simulink model "Simulaciones_Actuadores_Reales"  (R2026b)
settings: Solver=ode15s  StopTime=15  MaxStep=0.001
values from neighbouring files (symbols this model uses):
  alpha_Cu = 3.9e-3    (= 0.0039)    [coeficientes.m]
  b_eq = b_m + b_l/(r^2)    (= 2.19444444444e-05)    [coeficientes.m]
  C_ts = 0.818    [coeficientes.m]
  consigna_p = [0 0 0 0 0 0 0 0 0 0 0 0 ... (16001 elements, 16001x1)]    [perfil_lut.mat]    (also in suavizador_de_consigna.m = p_s(:))
  consigna_t = [0 0.001 0.002 0.003 0.004 0.005 0.006 0.007 0.008 0.009 0.01 0.011 ... (16001 elements, 16001x1)]    [perfil_lut.mat]    (also in suavizador_de_consigna.m = t(:))
  consigna_v = [0 0 0 0 0 0 0 0 0 0 0 0 ... (16001 elements, 16001x1)]    [perfil_lut.mat]    (also in suavizador_de_consigna.m = v_s(:))
  g = 9.80665    [coeficientes.m]
  init_I0 = 0    [coeficientes.m]
  init_Id = 0    [coeficientes.m]
  init_Iq = 0    [coeficientes.m]
  init_theta = 0    [coeficientes.m]
  init_Ts = 20    [coeficientes.m]
  init_w = 0    [coeficientes.m]
  J_eq = J_m + J_l/(r^2)    (= 4.58263888889e-05)    [coeficientes.m]
  K_et = 2*p_obs    (= 6400)    [coeficientes.m]
  K_ew = p_obs^2    (= 10240000)    [coeficientes.m]
  k_l = k_l_min + m_l*l_l    (= 1)    [coeficientes.m]
  Kd_mov = wn_mov * (2*zeta_mov + 1) * J_eq    (= 0.0916527777778)    [coeficientes.m]
  Ki_mov = wn_mov^3 * J_eq    (= 23463.1111111)    [coeficientes.m]
  Kp_mov = wn_mov^2 * (2*zeta_mov + 1) * J_eq    (= 73.3222222222)    [coeficientes.m]
  L_d = 6.6e-3    (= 0.0066)    [coeficientes.m]
  L_ls = 0.8e-3    (= 0.0008)    [coeficientes.m]
  L_q = 5.8e-3    (= 0.0058)    [coeficientes.m]
  lambda = 0.016    [coeficientes.m]
  Pp = 3    [coeficientes.m]
  r = 120.0    (= 120)    [coeficientes.m]
  R0 = abs(p)*L_ls    [coeficientes.m]
  R_sREF = 1.02    [coeficientes.m]
  R_tsamb = 146.7    [coeficientes.m]
  Rd = abs(p)*L_d    [coeficientes.m]
  Rq = abs(p)*L_q    [coeficientes.m]
  sat_V = sqrt(2/3)*V_slMAX    [coeficientes.m]
  T_amb = 20    [coeficientes.m]
  T_sREF = 20    [coeficientes.m]
  tau_RTD = %g s.\n',      base.wn_E,base.wn_I,base.wn_V,base.tau_RTD)    [barrido_filtros_reales.m]    (also in coeficientes.m = 20)
  wn_E = 6000    [coeficientes.m]
  wn_I = 2*6000    (= 12000)    [coeficientes.m]
  wn_V = 8500    [coeficientes.m]
  zeta_E = 1    [coeficientes.m]
  zeta_I = 1    [coeficientes.m]
  zeta_V = 1    [coeficientes.m]
libraries: eeTransforms x5
settings Model: Creator=fedeb  LastModifiedBy=fedeb
settings SimscapeCC: SimscapeLogType=all  SimscapeNominalValues="[{\"value\":\"1\",\"unit\":\"A\"},{\"value\":\"1\",\"unit\":\"bar\"},{\"value\":\"1\",\"unit\":\"cm^2\"},{\"value\":\"1\",\"unit\":\"cm^3/s\"},{\"value\":\"1\",\"unit\":\"kJ/kg\"},{\"value\":\"1\",\"unit\":\"kW\"},{\"value\":\"1\",\"unit\":\"l\"},{\"value\":\"1\",\"unit\":\"N\"},{\"value\":\"1\",\"unit\":\"N*m\"},{\"value\":\"1\",\"unit\":\"V\"},{\"value\":\"0.001\",\"unit\":\"Wb\"}]"  SimscapeUseEnergyAccounting=off

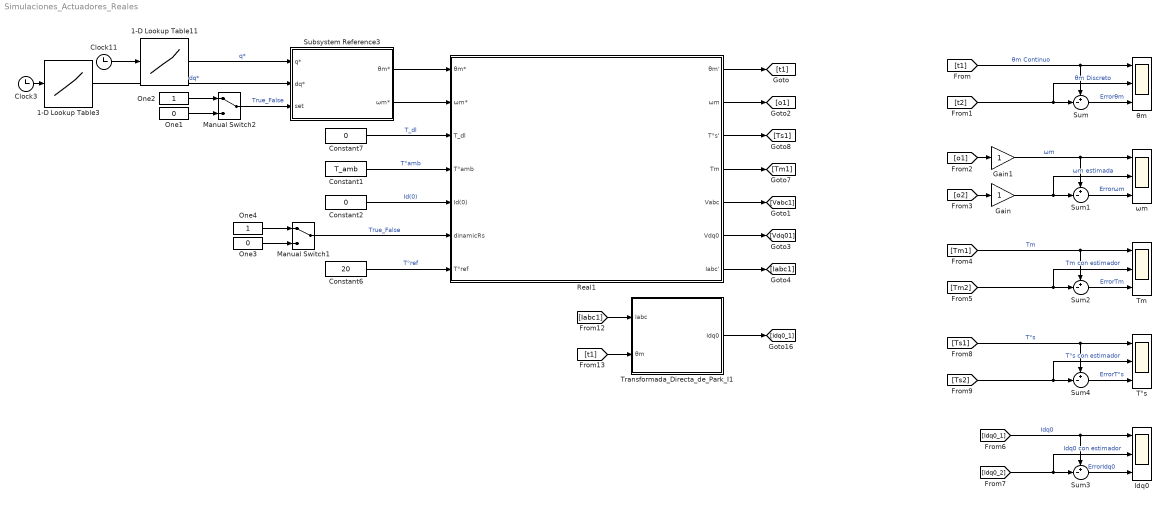
== system Simulaciones_Actuadores_Reales ==
  1-D Lookup Table11 : Lookup_n-D  NumberOfTableDimensions=1  BreakpointsForDimension1=consigna_t  Table=consigna_p  InternalRulePriority=Speed  RndMeth=Simplest
  1-D Lookup Table3 : Lookup_n-D  NumberOfTableDimensions=1  BreakpointsForDimension1=consigna_t  Table=consigna_v  InternalRulePriority=Speed  RndMeth=Simplest
  Clock11 : Clock
  Clock3 : Clock
  Constant1 : Constant  Value=T_amb
  Constant2 : Constant  Value=0
  Constant6 : Constant  Value=20
  Constant7 : Constant  Value=0
  Gain : Gain
  Gain1 : Gain
  Idq0 : Scope  NumInputPorts=3
      settings: Title=Comparación I0 con perturbación  ActiveDisplayYMinimum=-1.47623346288452  ActiveDisplayYMaximum=1.4762334392820955  YLabel=I0 [A]  DataLoggingVariableName=ScopeData3
  Manual Switch1 : ManualSwitch
  Manual Switch2 : ManualSwitch
  One1 : Constant  Value=0  OutDataTypeStr=Inherit: Inherit via back propagation
  One2 : Constant  OutDataTypeStr=Inherit: Inherit via back propagation
  One3 : Constant  Value=0  OutDataTypeStr=Inherit: Inherit via back propagation
  One4 : Constant  OutDataTypeStr=Inherit: Inherit via back propagation
  Real1 : Subsystem
  Subsystem Reference3 : Subsystem
  Sum{,1..4} (5 alike) : Sum  Inputs=+-|
  Tm : Scope  NumInputPorts=3
      settings: Title=Comparación Torque Motor con Perturbacion Tl  ActiveDisplayYMinimum=-0.10628903515783512  ActiveDisplayYMaximum=0.10628903470442332  YLabel=T_m [Nm]
  Transformada_Directa_de_Park_I1 : Subsystem
  T°s : Scope  NumInputPorts=3
      settings: Title=Comparación Temperatura del Estator con Perturbacion Tl  ActiveDisplayYMinimum=-3.1512581688392318  ActiveDisplayYMaximum=28.361323519553096  YLabel=T\circ  DataLoggingVariableName=ScopeData2
  θm : Scope  NumInputPorts=3
      settings: Title=Comparación θ motor con Perturbacion Tl  ActiveDisplayYMinimum=-94.247779700455553  ActiveDisplayYMaximum=848.23001656222721  YLabel=\theta_m[rad]  DataLoggingVariableName=ScopeData4
  ωm : Scope  NumInputPorts=3
      settings: Title=Comparación ωm con Perturbacion Tl  ActiveDisplayYMinimum=-188.49630294307897  ActiveDisplayYMaximum=188.49630291016143  YLabel=\omega_{motor} [10^3 rad/s]  DataLoggingVariableName=ScopeData5
  wires:
  Transformada_Directa_de_Park_I1/1(Idq0) -> [Idq0_1]
  Real1/4(Tm) -> [Tm1]
  Subsystem Reference3/2(ωm*) -> Real1/2(ωm*)
  Constant1/1 -> Real1/4(T°amb)  "T°amb"
  Constant6/1 -> Real1/7(T°ref)  "T°ref"
  Real1/3(T°s') -> [Ts1]
  [t1] -> θm/1, Sum/1  "θm Continuo"
  [Ts1] -> T°s/1, Sum4/1  "T°s"
  [t2] -> θm/2, Sum/2  "θm Discreto"
  Manual Switch2/1 -> Subsystem Reference3/3(set)  "True_False"
  [o2] -> Gain/1
  One3/1 -> Manual Switch1/2
  [Tm2] -> Tm/2, Sum2/2  "Tm con estimador"
  One1/1 -> Manual Switch2/2
  Real1/6(Vdq0) -> [Vdq01]
  Constant7/1 -> Real1/3(T_dl)  "T_dl"
  Gain/1 -> ωm/2, Sum1/2  "ωm estimada"
  Real1/1(θm') -> [t1]
  Subsystem Reference3/1(θm*) -> Real1/1(θm*)
  Real1/5(Vabc) -> [Vabc1]
  Clock3/1 -> 1-D Lookup Table3/1
  1-D Lookup Table11/1 -> Subsystem Reference3/1(q*)  "q*"
  Real1/2(ωm) -> [o1]
  Clock11/1 -> 1-D Lookup Table11/1
  [Ts2] -> T°s/2, Sum4/2  "T°s con estimador"
  Sum3/1 -> Idq0/3  "ErrorIdq0"
  1-D Lookup Table3/1 -> Subsystem Reference3/2(dq*)  "dq*"
  [Tm1] -> Tm/1, Sum2/1  "Tm"
  One2/1 -> Manual Switch2/1
  Sum4/1 -> T°s/3  "ErrorT°s"
  Constant2/1 -> Real1/5(Id(0))  "Id(0)"
  Sum2/1 -> Tm/3  "ErrorTm"
  [o1] -> Gain1/1
  [t1] -> Transformada_Directa_de_Park_I1/2(θm)
  Real1/7(Iabc') -> [Iabc1]
  [Idq0_2] -> Idq0/2, Sum3/2  "Idq0 con estimador"
  [Idq0_1] -> Sum3/1, Idq0/1  "Idq0"
  [Iabc1] -> Transformada_Directa_de_Park_I1/1(Iabc)
  Manual Switch1/1 -> Real1/6(dinamicRs)  "True_False"
  Sum/1 -> θm/3  "Errorθm"
  One4/1 -> Manual Switch1/1
  Sum1/1 -> ωm/3  "Errorωm"
  Gain1/1 -> ωm/1, Sum1/1  "ωm"

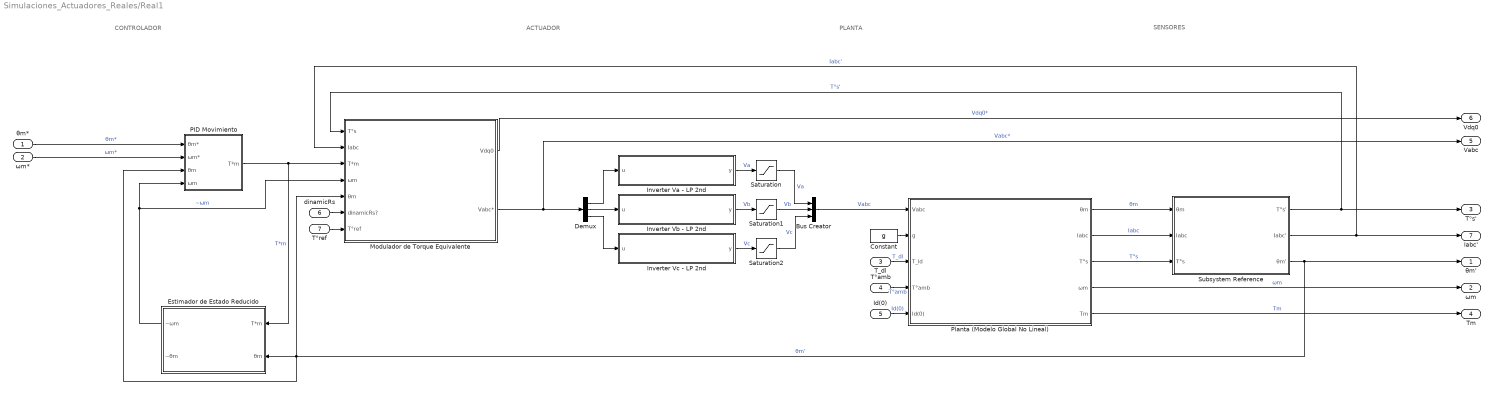
== system Simulaciones_Actuadores_Reales/Real1 ==
  note: ACTUADOR
  note: SENSORES
  note: CONTROLADOR
  note: PLANTA
  θm* : Inport
  ωm* : Inport  Port=2
  T_dl : Inport  Port=3
  T°amb : Inport  Port=4
  Id(0) : Inport  Port=5
  dinamicRs : Inport  Port=6
  T°ref : Inport  Port=7
  Bus Creator : BusCreator  Inputs=3
  Constant : Constant  Value=g
  Demux : Demux  Outputs=3
  Estimador de Estado Reducido : Subsystem
  Inverter Va - LP 2nd : Subsystem
  Inverter Vb - LP 2nd : Subsystem
  Inverter Vc - LP 2nd : Subsystem
  Modulador de Torque Equivalente : Subsystem
      settings: PortSchema="{\"entries\":[{\"content\":{\"sides\":[{\"content\":{\"connectorIds\":[\"In1\",\"In3\",\"In5\",\"In2\",\"In4\",\"In6\",\"In7\"]},\"type\":\"ConnectorPlacement.EquallySpacedRectSide\",\"uuid\":\"ea9ad4ab-f607-4d37-9442-85f6cfda2486\"},{\"content\":{\"connectorIds\":[\"Out2\",\"Out1\"],\"side\":\"RIGHT\"},\"type\":\"ConnectorPlacement.EquallySpacedRectSide\",\"uuid\":\"696b5fe5-1f6c-4fc9-932e-86b56d49996f\"},{\"content\":{\"side\":\"TOP\"},\"type\":\"ConnectorPlacement.EquallySpacedRectSide\",\"uuid\":\"45e3ac4c-5a2f-4a79-9454-e497b07295c7\"}]},\"type\":\"ConnectorPlacement.EquallySpacedConnector\",\"uuid\":\"ad401c21-3c60-4ab4-96eb-f449fc93609a\"}],\"packageUris\":[\"http://schema.mathworks.com/mf0/Connector/R2020b\"],\"version\":\"1.0\"}"
  PID Movimiento : Subsystem
      settings: PortSchema="{\"entries\":[{\"content\":{\"sides\":[{\"content\":{\"connectorIds\":[\"In3\",\"In4\",\"In2\",\"In1\"]},\"type\":\"ConnectorPlacement.EquallySpacedRectSide\",\"uuid\":\"99b9ec4b-f651-40ed-8a16-085c2c4ac88d\"},{\"content\":{\"connectorIds\":[\"Out1\"],\"side\":\"RIGHT\"},\"type\":\"ConnectorPlacement.EquallySpacedRectSide\",\"uuid\":\"009a9369-fd86-4ac2-a423-7c7f1491457b\"},{\"content\":{\"side\":\"TOP\"},\"type\":\"ConnectorPlacement.EquallySpacedRectSide\",\"uuid\":\"0bc889a5-9100-482e-a11a-4c36993d76f7\"}]},\"type\":\"ConnectorPlacement.EquallySpacedConnector\",\"uuid\":\"de270b8a-8a15-46e7-87f3-10db7988a399\"}],\"packageUris\":[\"http://schema.mathworks.com/mf0/Connector/R2020b\"],\"version\":\"1.0\"}"
  Planta (Modelo Global No Lineal) : Subsystem
      settings: PortSchema="{\"entries\":[{\"content\":{\"sides\":[{\"content\":{\"connectorIds\":[\"In1\",\"In3\",\"In2\",\"In4\",\"In5\"]},\"type\":\"ConnectorPlacement.EquallySpacedRectSide\",\"uuid\":\"3481abf0-b0cb-49f6-b93f-5a31fbfa4119\"},{\"content\":{\"connectorIds\":[\"Out1\",\"Out2\",\"Out3\",\"Out4\",\"Out5\"],\"side\":\"RIGHT\"},\"type\":\"ConnectorPlacement.EquallySpacedRectSide\",\"uuid\":\"81dbc61e-d5f3-4edc-bc73-ec3d6160a008\"},{\"content\":{\"side\":\"TOP\"},\"type\":\"ConnectorPlacement.EquallySpacedRectSide\",\"uuid\":\"48e37594-92fb-4835-b4aa-9211b8b6a309\"}]},\"type\":\"ConnectorPlacement.EquallySpacedConnector\",\"uuid\":\"6c32b8e1-5803-41f4-af4e-ba3a494349ba\"}],\"packageUris\":[\"http://schema.mathworks.com/mf0/Connector/R2020b\"],\"version\":\"1.0\"}"
  Saturation : Saturate  UpperLimit=sat_V  LowerLimit=-sat_V
  Saturation1 : Saturate  UpperLimit=sat_V  LowerLimit=-sat_V
  Saturation2 : Saturate  UpperLimit=sat_V  LowerLimit=-sat_V
  Subsystem Reference : Subsystem
  θm' : Outport
  ωm : Outport  Port=2
  T°s' : Outport  Port=3
  Tm : Outport  Port=4
  Vabc : Outport  Port=5  OutDataTypeStr=Bus: Vabc
  Vdq0 : Outport  Port=6  OutDataTypeStr=Bus: Vdq0
  Iabc' : Outport  Port=7  OutDataTypeStr=Bus: Iabc
  wires:
  Subsystem Reference/2(Iabc') -> Modulador de Torque Equivalente/3(Iabc), Iabc'/1  "Iabc'"
  Planta (Modelo Global No Lineal)/2(Iabc) -> Subsystem Reference/2(Iabc)  "Iabc"
  T°amb/1 -> Planta (Modelo Global No Lineal)/4(T°amb)  "T°amb"
  T°ref/1 -> Modulador de Torque Equivalente/7(T°ref)
  T_dl/1 -> Planta (Modelo Global No Lineal)/2(T_ld)  "T_dl"
  Subsystem Reference/1(T°s') -> Modulador de Torque Equivalente/1(T°s), T°s'/1  "T°s'"
  dinamicRs/1 -> Modulador de Torque Equivalente/6(dinamicRs?)
  Planta (Modelo Global No Lineal)/5(Tm) -> Tm/1  "Tm"
  θm*/1 -> PID Movimiento/3(θm*)  "θm*"
  Modulador de Torque Equivalente/2(Vdq0) -> Vdq0/1  "Vdq0*"
  Planta (Modelo Global No Lineal)/4(ωm) -> ωm/1  "ωm"
  PID Movimiento/1(T*m) -> Estimador de Estado Reducido/1(T*m), Modulador de Torque Equivalente/5(T*m)  "T*m"
  Estimador de Estado Reducido/1(~ωm) -> PID Movimiento/1(ωm), Modulador de Torque Equivalente/2(ωm)  "~ωm"
  Constant/1 -> Planta (Modelo Global No Lineal)/3(g)
  ωm*/1 -> PID Movimiento/4(ωm*)  "ωm*"
  Planta (Modelo Global No Lineal)/1(θm) -> Subsystem Reference/1(θm)  "θm"
  Id(0)/1 -> Planta (Modelo Global No Lineal)/5(Id(0))  "Id(0)"
  Subsystem Reference/3(θm') -> Modulador de Torque Equivalente/4(θm), PID Movimiento/2(θm), Estimador de Estado Reducido/2(θm), θm'/1  "θm'"
  Planta (Modelo Global No Lineal)/3(T°s) -> Subsystem Reference/3(T°s)  "T°s"
  Demux/2 -> Inverter Vb - LP 2nd/1(u)
  Inverter Vc - LP 2nd/1(y) -> Saturation2/1  "Vc"
  Saturation1/1 -> Bus Creator/2  "Vb"
  Inverter Vb - LP 2nd/1(y) -> Saturation1/1  "Vb"
  Demux/1 -> Inverter Va - LP 2nd/1(u)
  Inverter Va - LP 2nd/1(y) -> Saturation/1  "Va"
  Demux/3 -> Inverter Vc - LP 2nd/1(u)
  Modulador de Torque Equivalente/1(Vabc*) -> Demux/1, Vabc/1  "Vabc*"
  Saturation2/1 -> Bus Creator/3  "Vc"
  Bus Creator/1 -> Planta (Modelo Global No Lineal)/1(Vabc)  "Vabc"
  Saturation/1 -> Bus Creator/1  "Va"

== system Simulaciones_Actuadores_Reales/Subsystem Reference3 ==
  q* : Inport
  dq* : Inport  Port=2
  set : Inport  Port=3
  Gain : Gain  Gain=r
  Gain1 : Gain  Gain=r
  Integrator : Integrator  ExternalReset=level  InitialConditionSource=external
  Selector : RelationalOperator  Operator=>  OutDataTypeStr=boolean  RndMeth=Simplest  InputSameDT=off
  Switch : Switch  Criteria=u2 ~= 0  SaturateOnIntegerOverflow=off  InputSameDT=off
  Umbral : Constant  Value=0.5
  θm* : Outport
  ωm* : Outport  Port=2
  wires:
  q*/1 -> Gain/1
  dq*/1 -> Gain1/1
  set/1 -> Selector/1
  Umbral/1 -> Selector/2
  Gain/1 -> Integrator/3, Switch/1
  Selector/1 -> Integrator/2, Switch/2
  Gain1/1 -> Integrator/1, ωm*/1
  Integrator/1 -> Switch/3
  Switch/1 -> θm*/1

== system Simulaciones_Actuadores_Reales/Transformada_Directa_de_Park_I1 ==
  Iabc : Inport  OutDataTypeStr=Bus: Iabc
  θm : Inport  Port=2
  Ancho_abc : SignalSpecification  Dimensions=3
  Bus Creator : BusCreator  Inputs=3
  Bus to Vector : BusToVector
  Demux : Demux  Outputs=3
  Gain3 : Gain  Gain=Pp
  Park Transform : eeTransforms/Park Transform  AxisAlignment=Q-axis  PowerInvariant=off
      settings: LibrarySourceBlock=|
      | ee_sl_lib/Mathematical
      | Transforms/Park Transform
  Idq0 : Outport  OutDataTypeStr=Bus: Idq0
  wires:
  Gain3/1 -> Park Transform/2
  Park Transform/1 -> Demux/1  "Idq0"
  Demux/1 -> Bus Creator/1  "Id"
  Demux/3 -> Bus Creator/3  "I0"
  Demux/2 -> Bus Creator/2  "Iq"
  Bus Creator/1 -> Idq0/1
  Iabc/1 -> Bus to Vector/1
  θm/1 -> Gain3/1
  Bus to Vector/1 -> Ancho_abc/1
  Ancho_abc/1 -> Park Transform/1

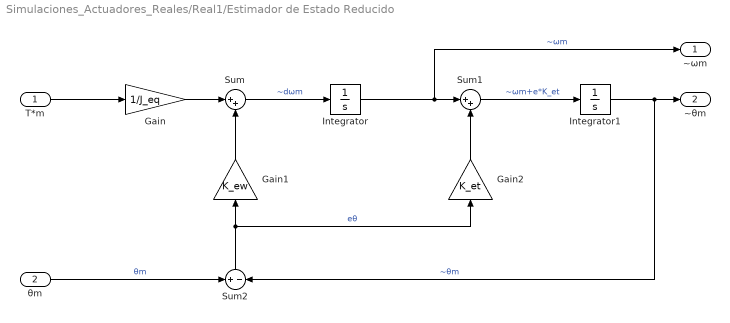
== system Simulaciones_Actuadores_Reales/Real1/Estimador de Estado Reducido ==
  T*m : Inport
  θm : Inport  Port=2
  Gain : Gain  Gain=1/J_eq
  Gain1 : Gain  Gain=K_ew
  Gain2 : Gain  Gain=K_et
  Integrator : Integrator
  Integrator1 : Integrator
  Sum : Sum  Inputs=|++
  Sum1 : Sum  Inputs=|++
  Sum2 : Sum  Inputs=+-
  ~ωm : Outport
  ~θm : Outport  Port=2
  wires:
  Integrator1/1 -> ~θm/1, Sum2/2  "~θm"
  θm/1 -> Sum2/1  "θm"
  Sum2/1 -> Gain2/1, Gain1/1  "eθ"
  Gain2/1 -> Sum1/2
  Gain1/1 -> Sum/2
  Integrator/1 -> Sum1/1, ~ωm/1  "~ωm"
  Sum1/1 -> Integrator1/1  "~ωm+e*K_et"
  Sum/1 -> Integrator/1  "~dωm"
  Gain/1 -> Sum/1
  T*m/1 -> Gain/1

== system Simulaciones_Actuadores_Reales/Real1/Inverter Va - LP 2nd ==
  u : Inport
  Gain : Gain  Gain=wn_V^2
  Gain1 : Gain  Gain=wn_V^2
  Gain2 : Gain  Gain=2*zeta_V*wn_V
  Integrator : Integrator
  Integrator1 : Integrator
  Sum : Sum  Inputs=|++
  Sum1 : Sum  Inputs=|+-
  y : Outport
  wires:
  u/1 -> Gain/1
  Gain/1 -> Sum1/1
  Sum/1 -> Sum1/2
  Sum1/1 -> Integrator/1
  Gain2/1 -> Sum/2
  Gain1/1 -> Sum/1
  Integrator/1 -> Gain2/1, Integrator1/1
  Integrator1/1 -> Gain1/1, y/1

== system Simulaciones_Actuadores_Reales/Real1/Inverter Vb - LP 2nd ==
  u : Inport
  Gain : Gain  Gain=wn_V^2
  Gain1 : Gain  Gain=wn_V^2
  Gain2 : Gain  Gain=2*zeta_V*wn_V
  Integrator : Integrator
  Integrator1 : Integrator
  Sum : Sum  Inputs=|++
  Sum1 : Sum  Inputs=|+-
  y : Outport
  wires:
  Integrator1/1 -> y/1, Gain1/1
  Integrator/1 -> Integrator1/1, Gain2/1
  Gain1/1 -> Sum/1
  Gain2/1 -> Sum/2
  Sum1/1 -> Integrator/1
  Sum/1 -> Sum1/2
  Gain/1 -> Sum1/1
  u/1 -> Gain/1

== system Simulaciones_Actuadores_Reales/Real1/Inverter Vc - LP 2nd ==
  u : Inport
  Gain : Gain  Gain=wn_V^2
  Gain1 : Gain  Gain=wn_V^2
  Gain2 : Gain  Gain=2*zeta_V*wn_V
  Integrator : Integrator
  Integrator1 : Integrator
  Sum : Sum  Inputs=|++
  Sum1 : Sum  Inputs=|+-
  y : Outport
  wires:
  u/1 -> Gain/1
  Gain/1 -> Sum1/1
  Sum/1 -> Sum1/2
  Sum1/1 -> Integrator/1
  Gain2/1 -> Sum/2
  Gain1/1 -> Sum/1
  Integrator/1 -> Gain2/1, Integrator1/1
  Integrator1/1 -> Gain1/1, y/1

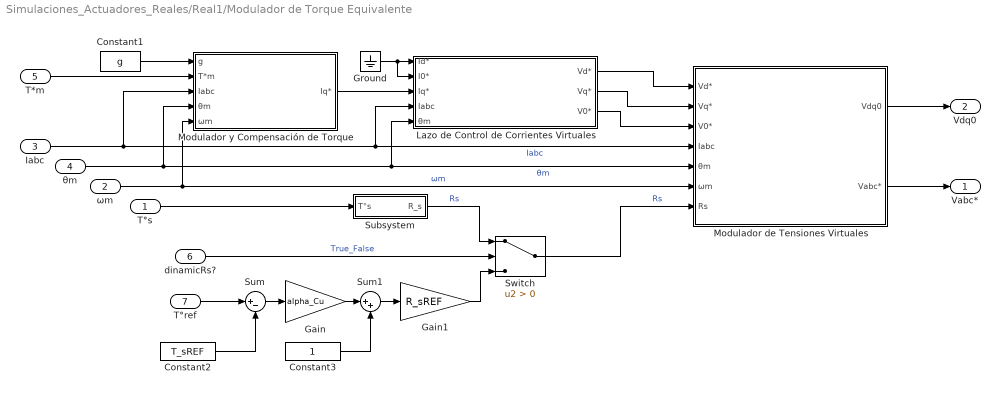
== system Simulaciones_Actuadores_Reales/Real1/Modulador de Torque Equivalente ==
  T°s : Inport
  ωm : Inport  Port=2
  Iabc : Inport  Port=3
  θm : Inport  Port=4
  T*m : Inport  Port=5
  dinamicRs? : Inport  Port=6
  T°ref : Inport  Port=7
  Constant1 : Constant  Value=g
  Constant2 : Constant  Value=T_sREF
  Constant3 : Constant
  Gain : Gain  Gain=alpha_Cu
  Gain1 : Gain  Gain=R_sREF
  Ground : Ground
  Lazo de Control de Corrientes Virtuales : Subsystem
      settings: PortSchema="{\"entries\":[{\"content\":{\"sides\":[{\"content\":{\"connectorIds\":[\"In2\",\"In3\",\"In1\",\"In4\",\"In5\"]},\"type\":\"ConnectorPlacement.EquallySpacedRectSide\",\"uuid\":\"7378df2b-1b9c-42cd-9ef6-9bfa4de31228\"},{\"content\":{\"connectorIds\":[\"Out2\",\"Out1\",\"Out3\"],\"side\":\"RIGHT\"},\"type\":\"ConnectorPlacement.EquallySpacedRectSide\",\"uuid\":\"75ac4e09-b611-4ee2-aa1e-16791f3f98b8\"},{\"content\":{\"side\":\"TOP\"},\"type\":\"ConnectorPlacement.EquallySpacedRectSide\",\"uuid\":\"c32b7829-5b6a-417b-8aae-eaa4caf59bef\"}]},\"type\":\"ConnectorPlacement.EquallySpacedConnector\",\"uuid\":\"1d84f5ff-db01-492a-bfe1-22065b3eebb0\"}],\"packageUris\":[\"http://schema.mathworks.com/mf0/Connector/R2020b\"],\"version\":\"1.0\"}"
  Modulador de Tensiones Virtuales : Subsystem
      settings: PortSchema="{\"entries\":[{\"content\":{\"sides\":[{\"content\":{\"connectorIds\":[\"In2\",\"In1\",\"In3\",\"In6\",\"In7\",\"In5\",\"In4\"]},\"type\":\"ConnectorPlacement.EquallySpacedRectSide\",\"uuid\":\"561a625a-719f-47d4-85d3-a88e423068dd\"},{\"content\":{\"connectorIds\":[\"Out2\",\"Out1\"],\"side\":\"RIGHT\"},\"type\":\"ConnectorPlacement.EquallySpacedRectSide\",\"uuid\":\"c1cdd74a-6c1d-470e-a6ac-8d72e83b5cc5\"},{\"content\":{\"side\":\"TOP\"},\"type\":\"ConnectorPlacement.EquallySpacedRectSide\",\"uuid\":\"c5935c6f-534c-46b9-aa64-6d6dabbbb210\"}]},\"type\":\"ConnectorPlacement.EquallySpacedConnector\",\"uuid\":\"b0debde9-6e18-4e06-b0c4-28c9c51e472d\"}],\"packageUris\":[\"http://schema.mathworks.com/mf0/Connector/R2020b\"],\"version\":\"1.0\"}"
  Modulador y Compensación de Torque : Subsystem
      settings: PortSchema="{\"entries\":[{\"content\":{\"sides\":[{\"content\":{\"connectorIds\":[\"In5\",\"In1\",\"In2\",\"In3\",\"In4\"]},\"type\":\"ConnectorPlacement.EquallySpacedRectSide\",\"uuid\":\"ea9ad4ab-f607-4d37-9442-85f6cfda2486\"},{\"content\":{\"connectorIds\":[\"Out1\"],\"side\":\"RIGHT\"},\"type\":\"ConnectorPlacement.EquallySpacedRectSide\",\"uuid\":\"696b5fe5-1f6c-4fc9-932e-86b56d49996f\"},{\"content\":{\"side\":\"TOP\"},\"type\":\"ConnectorPlacement.EquallySpacedRectSide\",\"uuid\":\"45e3ac4c-5a2f-4a79-9454-e497b07295c7\"}]},\"type\":\"ConnectorPlacement.EquallySpacedConnector\",\"uuid\":\"ad401c21-3c60-4ab4-96eb-f449fc93609a\"}],\"packageUris\":[\"http://schema.mathworks.com/mf0/Connector/R2020b\"],\"version\":\"1.0\"}"
  Subsystem : Subsystem
  Sum : Sum  Inputs=|+-
  Sum1 : Sum  Inputs=|++
  Switch : Switch  Criteria=u2 > Threshold  SaturateOnIntegerOverflow=off  InputSameDT=off
  Vabc* : Outport
  Vdq0 : Outport  Port=2
  wires:
  Sum1/1 -> Gain1/1
  Constant3/1 -> Sum1/2
  Gain/1 -> Sum1/1
  Sum/1 -> Gain/1
  Constant2/1 -> Sum/2
  T°ref/1 -> Sum/1
  Constant1/1 -> Modulador y Compensación de Torque/5(g)
  Modulador de Tensiones Virtuales/2(Vdq0) -> Vdq0/1
  Gain1/1 -> Switch/3
  Switch/1 -> Modulador de Tensiones Virtuales/4(Rs)  "Rs"
  dinamicRs?/1 -> Switch/2  "True_False"
  Subsystem/1(R_s) -> Switch/1  "Rs"
  T°s/1 -> Subsystem/1(T°s)
  Iabc/1 -> Modulador y Compensación de Torque/2(Iabc), Lazo de Control de Corrientes Virtuales/4(Iabc), Modulador de Tensiones Virtuales/6(Iabc)  "Iabc"
  Ground/1 -> Lazo de Control de Corrientes Virtuales/3(I0*), Lazo de Control de Corrientes Virtuales/2(Id*)
  Modulador de Tensiones Virtuales/1(Vabc*) -> Vabc*/1
  ωm/1 -> Modulador y Compensación de Torque/4(ωm), Modulador de Tensiones Virtuales/5(ωm)  "ωm"
  θm/1 -> Modulador y Compensación de Torque/3(θm), Lazo de Control de Corrientes Virtuales/5(θm), Modulador de Tensiones Virtuales/7(θm)  "θm"
  T*m/1 -> Modulador y Compensación de Torque/1(T*m)
  Modulador y Compensación de Torque/1(Iq*) -> Lazo de Control de Corrientes Virtuales/1(Iq*)
  Lazo de Control de Corrientes Virtuales/3(V0*) -> Modulador de Tensiones Virtuales/3(V0*)
  Lazo de Control de Corrientes Virtuales/2(Vd*) -> Modulador de Tensiones Virtuales/2(Vd*)
  Lazo de Control de Corrientes Virtuales/1(Vq*) -> Modulador de Tensiones Virtuales/1(Vq*)

== system Simulaciones_Actuadores_Reales/Real1/PID Movimiento ==
  ωm : Inport  Unit=rad/s
  θm : Inport  Port=2
  θm* : Inport  Port=3  Unit=rad/s
  ωm* : Inport  Port=4  Unit=rad/s
  Gain : Gain  Gain=Kd_mov
  Gain1 : Gain  Gain=Kp_mov
  Gain2 : Gain  Gain=Ki_mov
  Integrator : Integrator
  Sum : Sum  Inputs=|+-
  Sum1 : Sum  Inputs=+++
  Sum2 : Sum  Inputs=|+-
  T*m : Outport
  wires:
  Sum2/1 -> Integrator/1, Gain1/1  "eθ"
  Integrator/1 -> Gain2/1  "e∫θ"
  ωm/1 -> Sum/2
  ωm*/1 -> Sum/1
  θm/1 -> Sum2/2
  Sum/1 -> Gain/1  "eω"
  θm*/1 -> Sum2/1
  Gain/1 -> Sum1/3
  Gain2/1 -> Sum1/1
  Sum1/1 -> T*m/1
  Gain1/1 -> Sum1/2

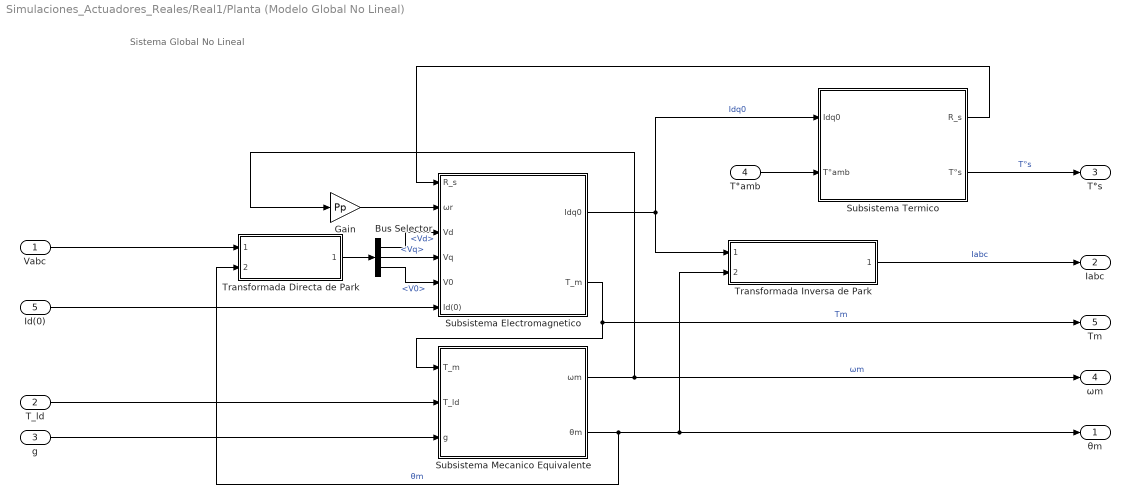
== system Simulaciones_Actuadores_Reales/Real1/Planta (Modelo Global No Lineal) ==
  note: Sistema Global No Lineal
  Vabc : Inport  OutDataTypeStr=Bus: Vabc
  T_ld : Inport  Port=2
  g : Inport  Port=3
  T°amb : Inport  Port=4
  Id(0) : Inport  Port=5
  Bus Selector : BusSelector  OutputSignals=Vd,Vq,V0
  Gain : Gain  Gain=Pp
  Subsistema Electromagnetico : Subsystem
  Subsistema Mecanico Equivalente : Subsystem
  Subsistema Termico : Subsystem
  Transformada Directa de Park : Subsystem  ReferencedSubsystem=Transformada_Directa_de_Park_V
  Transformada Inversa de Park : Subsystem  ReferencedSubsystem=Transformada_Inversa_de_Park_I
  θm : Outport
  Iabc : Outport  Port=2  OutDataTypeStr=Bus: Iabc
  T°s : Outport  Port=3
  ωm : Outport  Port=4
  Tm : Outport  Port=5
  wires:
  Id(0)/1 -> Subsistema Electromagnetico/6(Id(0))
  Transformada Inversa de Park/1 -> Iabc/1  "Iabc"
  Bus Selector/3 -> Subsistema Electromagnetico/5(V0)  "<V0>"
  Bus Selector/2 -> Subsistema Electromagnetico/4(Vq)  "<Vq>"
  Bus Selector/1 -> Subsistema Electromagnetico/3(Vd)  "<Vd>"
  Transformada Directa de Park/1 -> Bus Selector/1
  g/1 -> Subsistema Mecanico Equivalente/3(g)
  T°amb/1 -> Subsistema Termico/2(T°amb)
  Vabc/1 -> Transformada Directa de Park/1
  T_ld/1 -> Subsistema Mecanico Equivalente/2(T_ld)
  Gain/1 -> Subsistema Electromagnetico/2(ωr)
  Subsistema Termico/1(R_s) -> Subsistema Electromagnetico/1(R_s)
  Subsistema Electromagnetico/2(T_m) -> Tm/1, Subsistema Mecanico Equivalente/1(T_m)  "Tm"
  Subsistema Mecanico Equivalente/2(θm) -> θm/1, Transformada Inversa de Park/2, Transformada Directa de Park/2  "θm"
  Subsistema Mecanico Equivalente/1(ωm) -> ωm/1, Gain/1  "ωm"
  Subsistema Electromagnetico/1(Idq0) -> Transformada Inversa de Park/1, Subsistema Termico/1(Idq0)  "Idq0"
  Subsistema Termico/2(T°s) -> T°s/1  "T°s"

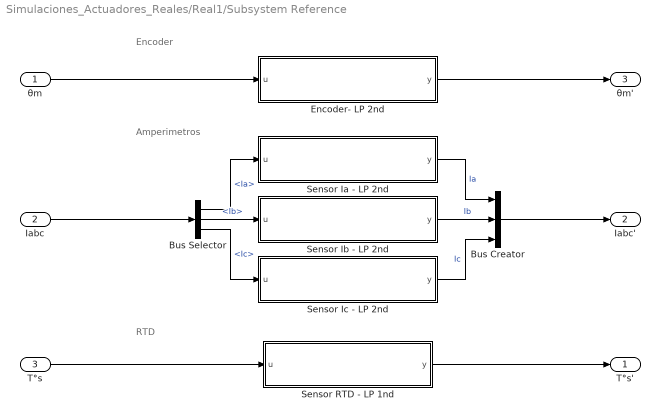
== system Simulaciones_Actuadores_Reales/Real1/Subsystem Reference ==
  note: Amperimetros
  note: Encoder
  note: RTD
  θm : Inport
  Iabc : Inport  Port=2
  T°s : Inport  Port=3
  Bus Creator : BusCreator  Inputs=3
  Bus Selector : BusSelector  OutputSignals=Ia,Ib,Ic
  Encoder- LP 2nd : Subsystem
  Sensor Ia - LP 2nd : Subsystem
  Sensor Ib - LP 2nd : Subsystem
  Sensor Ic - LP 2nd : Subsystem
  Sensor RTD - LP 1nd : Subsystem
  T°s' : Outport
  Iabc' : Outport  Port=2
  θm' : Outport  Port=3
  wires:
  Sensor Ib - LP 2nd/1(y) -> Bus Creator/2  "Ib"
  Sensor RTD - LP 1nd/1(y) -> T°s'/1
  Sensor Ia - LP 2nd/1(y) -> Bus Creator/1  "Ia"
  Bus Creator/1 -> Iabc'/1
  Encoder- LP 2nd/1(y) -> θm'/1
  Bus Selector/1 -> Sensor Ia - LP 2nd/1(u)  "<Ia>"
  Bus Selector/2 -> Sensor Ib - LP 2nd/1(u)  "<Ib>"
  T°s/1 -> Sensor RTD - LP 1nd/1(u)
  Bus Selector/3 -> Sensor Ic - LP 2nd/1(u)  "<Ic>"
  Iabc/1 -> Bus Selector/1
  θm/1 -> Encoder- LP 2nd/1(u)
  Sensor Ic - LP 2nd/1(y) -> Bus Creator/3  "Ic"

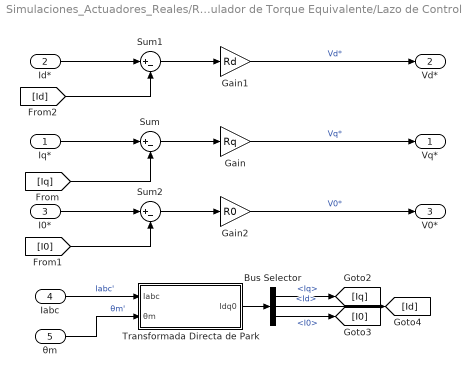
== system Simulaciones_Actuadores_Reales/Real1/Modulador de Torque Equivalente/Lazo de Control de Corrientes Virtuales ==
  Iq* : Inport
  Id* : Inport  Port=2
  I0* : Inport  Port=3
  Iabc : Inport  Port=4
  θm : Inport  Port=5
  Bus Selector : BusSelector  OutputSignals=Iq,Id,I0
  Gain : Gain  Gain=Rq
  Gain1 : Gain  Gain=Rd
  Gain2 : Gain  Gain=R0
  Sum : Sum  Inputs=|+-
  Sum1 : Sum  Inputs=|+-
  Sum2 : Sum  Inputs=|+-
  Transformada Directa de Park : Subsystem
  Vq* : Outport
  Vd* : Outport  Port=2
  V0* : Outport  Port=3
  wires:
  Sum1/1 -> Gain1/1
  Gain/1 -> Vq*/1  "Vq*"
  Id*/1 -> Sum1/1
  Iq*/1 -> Sum/1
  Gain1/1 -> Vd*/1  "Vd*"
  [Iq] -> Sum/2
  [Id] -> Sum1/2
  Sum/1 -> Gain/1
  Gain2/1 -> V0*/1  "V0*"
  Sum2/1 -> Gain2/1
  [I0] -> Sum2/2
  I0*/1 -> Sum2/1
  Bus Selector/2 -> [Id]  "<Id>"
  Bus Selector/3 -> [I0]  "<I0>"
  Transformada Directa de Park/1(Idq0) -> Bus Selector/1
  Iabc/1 -> Transformada Directa de Park/1(Iabc)  "Iabc'"
  θm/1 -> Transformada Directa de Park/2(θm)  "θm'"
  Bus Selector/1 -> [Iq]  "<Iq>"

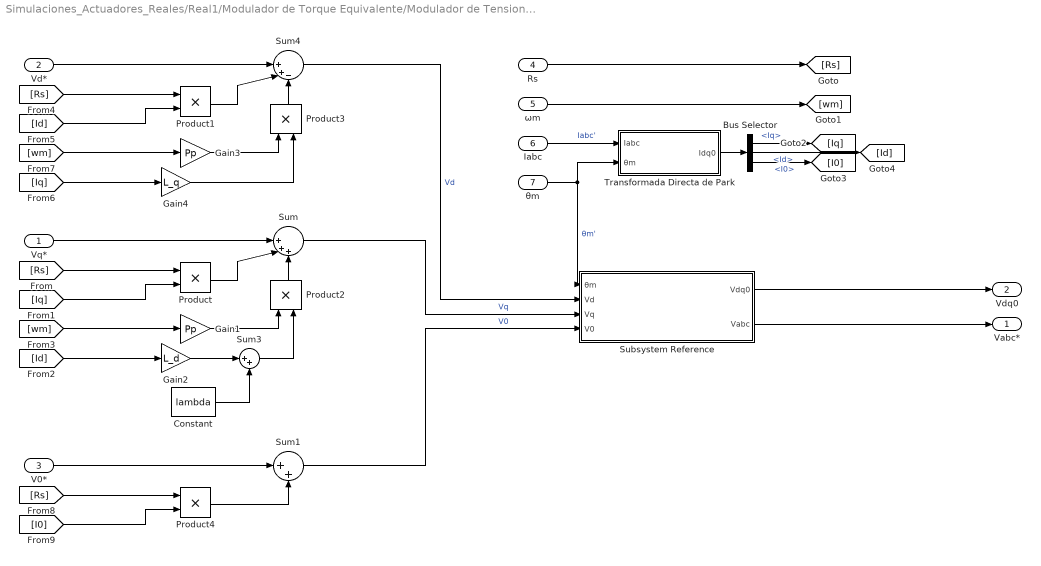
== system Simulaciones_Actuadores_Reales/Real1/Modulador de Torque Equivalente/Modulador de Tensiones Virtuales ==
  Vq* : Inport
  Vd* : Inport  Port=2
  V0* : Inport  Port=3
  Rs : Inport  Port=4
  ωm : Inport  Port=5
  Iabc : Inport  Port=6
  θm : Inport  Port=7
  Bus Selector : BusSelector  OutputSignals=Iq,Id,I0
  Constant : Constant  Value=lambda
  Gain1 : Gain  Gain=Pp
  Gain2 : Gain  Gain=L_d
  Gain3 : Gain  Gain=Pp
  Gain4 : Gain  Gain=L_q
  Product{,1..4} (5 alike) : Product
  Subsystem Reference : Subsystem
  Sum : Sum  Inputs=||+++
  Sum1 : Sum  Inputs=|++
  Sum3 : Sum  Inputs=|++
  Sum4 : Sum  Inputs=||++-
  Transformada Directa de Park : Subsystem
  Vabc* : Outport
  Vdq0 : Outport  Port=2
  wires:
  Sum1/1 -> Subsystem Reference/4(V0)  "V0"
  Sum/1 -> Subsystem Reference/3(Vq)  "Vq"
  Sum4/1 -> Subsystem Reference/2(Vd)  "Vd"
  Subsystem Reference/1(Vdq0) -> Vdq0/1
  Iabc/1 -> Transformada Directa de Park/1(Iabc)  "Iabc'"
  Transformada Directa de Park/1(Idq0) -> Bus Selector/1
  θm/1 -> Transformada Directa de Park/2(θm), Subsystem Reference/1(θm)  "θm'"
  Subsystem Reference/2(Vabc) -> Vabc*/1
  Rs/1 -> [Rs]
  ωm/1 -> [wm]
  Bus Selector/1 -> [Iq]  "<Iq>"
  Bus Selector/3 -> [I0]  "<I0>"
  Bus Selector/2 -> [Id]  "<Id>"
  Vq*/1 -> Sum/1
  [Rs] -> Product/1
  Product/1 -> Sum/2
  Constant/1 -> Sum3/2
  [Id] -> Gain2/1
  Gain2/1 -> Sum3/1
  Product2/1 -> Sum/3
  [wm] -> Gain1/1
  Sum3/1 -> Product2/2
  Gain1/1 -> Product2/1
  [Iq] -> Product/2
  [wm] -> Gain3/1
  Product1/1 -> Sum4/2
  [Iq] -> Gain4/1
  Gain3/1 -> Product3/1
  [Rs] -> Product1/1
  Vd*/1 -> Sum4/1
  Gain4/1 -> Product3/2
  Product3/1 -> Sum4/3
  [Id] -> Product1/2
  [I0] -> Product4/2
  [Rs] -> Product4/1
  V0*/1 -> Sum1/1
  Product4/1 -> Sum1/2

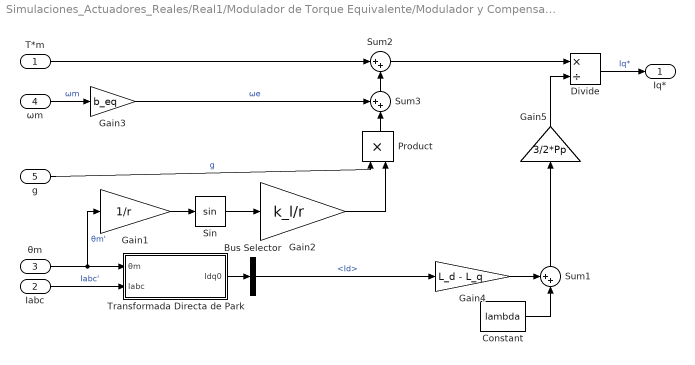
== system Simulaciones_Actuadores_Reales/Real1/Modulador de Torque Equivalente/Modulador y Compensación de Torque ==
  T*m : Inport
  Iabc : Inport  Port=2
  θm : Inport  Port=3
  ωm : Inport  Port=4
  g : Inport  Port=5
  Bus Selector : BusSelector  OutputSignals=Id
  Constant : Constant  Value=lambda
  Divide : Product  Inputs=*/
  Gain1 : Gain  Gain=1/r
  Gain2 : Gain  Gain=k_l/r
  Gain3 : Gain  Gain=b_eq
  Gain4 : Gain  Gain=L_d - L_q
  Gain5 : Gain  Gain=3/2*Pp
  Product : Product
  Sin : Trigonometry
  Sum1 : Sum  Inputs=++|
  Sum2 : Sum  Inputs=|++
  Sum3 : Sum  Inputs=++|
  Transformada Directa de Park : Subsystem
  Iq* : Outport
  wires:
  Sum3/1 -> Sum2/2
  Gain3/1 -> Sum3/1  "ωe"
  ωm/1 -> Gain3/1  "ωm"
  g/1 -> Product/1  "g"
  Gain2/1 -> Product/2
  Product/1 -> Sum3/2
  Sin/1 -> Gain2/1
  Gain1/1 -> Sin/1
  Bus Selector/1 -> Gain4/1  "<Id>"
  Gain5/1 -> Divide/2
  Sum2/1 -> Divide/1
  Sum1/1 -> Gain5/1
  Constant/1 -> Sum1/2
  Gain4/1 -> Sum1/1
  Transformada Directa de Park/1(Idq0) -> Bus Selector/1
  θm/1 -> Transformada Directa de Park/1(θm), Gain1/1  "θm'"
  Iabc/1 -> Transformada Directa de Park/2(Iabc)  "Iabc'"
  T*m/1 -> Sum2/1
  Divide/1 -> Iq*/1  "Iq*"

== system Simulaciones_Actuadores_Reales/Real1/Modulador de Torque Equivalente/Subsystem ==
  T°s : Inport
  Constant1 : Constant  Value=T_sREF
  Constant2 : Constant
  Gain5 : Gain  Gain=alpha_Cu
  Gain6 : Gain  Gain=R_sREF
  Sum3 : Sum  Inputs=+-|
  Sum4 : Sum  Inputs=|++
  R_s : Outport
  wires:
  Sum3/1 -> Gain5/1
  Sum4/1 -> Gain6/1
  Constant2/1 -> Sum4/2
  Constant1/1 -> Sum3/2
  Gain6/1 -> R_s/1  "R_s"
  Gain5/1 -> Sum4/1
  T°s/1 -> Sum3/1

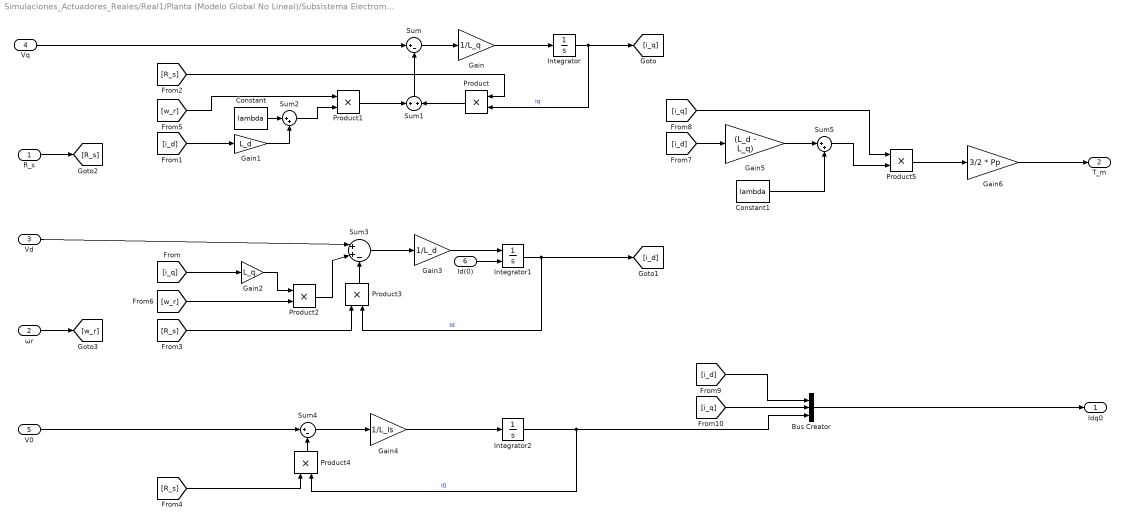
== system Simulaciones_Actuadores_Reales/Real1/Planta (Modelo Global No Lineal)/Subsistema Electromagnetico ==
  R_s : Inport
  ωr : Inport  Port=2
  Vd : Inport  Port=3
  Vq : Inport  Port=4
  V0 : Inport  Port=5
  Id(0) : Inport  Port=6
  Bus Creator : BusCreator  Inputs=3
  Constant : Constant  Value=lambda
  Constant1 : Constant  Value=lambda
  Gain : Gain  Gain=1/L_q
  Gain1 : Gain  Gain=L_d
  Gain2 : Gain  Gain=L_q
  Gain3 : Gain  Gain=1/L_d
  Gain4 : Gain  Gain=1/L_ls
  Gain5 : Gain  Gain=(L_d - L_q)
  Gain6 : Gain  Gain=3/2 * Pp
  Integrator : Integrator  InitialCondition=init_Iq
  Integrator1 : Integrator  InitialConditionSource=external  InitialCondition=init_Id
  Integrator2 : Integrator  InitialCondition=init_I0
  Product{,1..5} (6 alike) : Product
  Sum : Sum  Inputs=|+-
  Sum1 : Sum
  Sum2 : Sum  Inputs=|++
  Sum3 : Sum  Inputs=|++-
  Sum4 : Sum  Inputs=|+-
  Sum5 : Sum  Inputs=|++
  Idq0 : Outport
  T_m : Outport  Port=2
  wires:
  [i_q] -> Bus Creator/2
  [i_d] -> Bus Creator/1
  Id(0)/1 -> Integrator1/2
  Bus Creator/1 -> Idq0/1
  [i_q] -> Product5/1
  [i_d] -> Gain5/1
  [w_r] -> Product1/1
  ωr/1 -> [w_r]
  [R_s] -> Product4/1
  [R_s] -> Product3/1
  R_s/1 -> [R_s]
  [i_d] -> Gain1/1
  Gain6/1 -> T_m/1
  Product5/1 -> Gain6/1
  Constant1/1 -> Sum5/2
  Integrator1/1 -> Product3/2, [i_d]  "Id"
  Sum5/1 -> Product5/2
  Gain5/1 -> Sum5/1
  V0/1 -> Sum4/1
  Sum4/1 -> Gain4/1
  Gain4/1 -> Integrator2/1
  Integrator2/1 -> Product4/2, Bus Creator/3  "I0"
  Product4/1 -> Sum4/2
  Vd/1 -> Sum3/1
  Sum3/1 -> Gain3/1
  Gain3/1 -> Integrator1/1
  Product3/1 -> Sum3/3
  Gain/1 -> Integrator/1
  Vq/1 -> Sum/1
  Sum/1 -> Gain/1
  Constant/1 -> Sum2/1
  Sum2/1 -> Product1/2
  Gain1/1 -> Sum2/2
  Product1/1 -> Sum1/1
  Sum1/1 -> Sum/2
  Product/1 -> Sum1/2
  [R_s] -> Product/1
  Integrator/1 -> [i_q], Product/2  "Iq"
  [i_q] -> Gain2/1
  Product2/1 -> Sum3/2
  Gain2/1 -> Product2/1
  [w_r] -> Product2/2

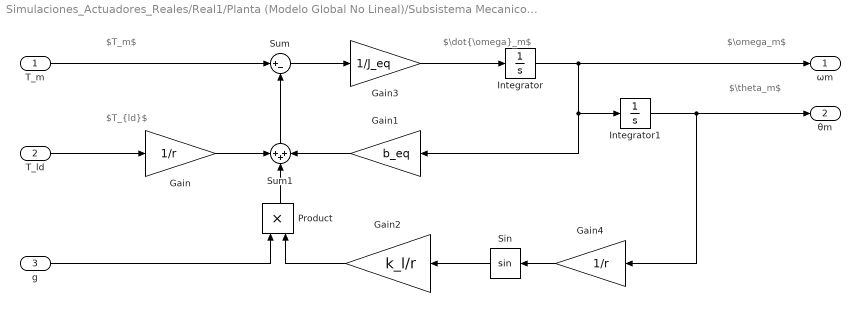
== system Simulaciones_Actuadores_Reales/Real1/Planta (Modelo Global No Lineal)/Subsistema Mecanico Equivalente ==
  note: $\theta_m$
  note: $\omega_m$
  note: $\dot{\omega}_m$
  note: $T_{ld}$
  note: $T_m$
  T_m : Inport
  T_ld : Inport  Port=2
  g : Inport  Port=3
  Gain : Gain  Gain=1/r
  Gain1 : Gain  Gain=b_eq
  Gain2 : Gain  Gain=k_l/r
  Gain3 : Gain  Gain=1/J_eq
  Gain4 : Gain  Gain=1/r
  Integrator : Integrator  InitialCondition=init_w
  Integrator1 : Integrator  InitialCondition=init_theta
  Product : Product
  Sin : Trigonometry
  Sum : Sum  Inputs=|+-
  Sum1 : Sum  Inputs=+++
  ωm : Outport
  θm : Outport  Port=2
  wires:
  Integrator1/1 -> θm/1, Gain4/1
  Integrator/1 -> Gain1/1, Integrator1/1, ωm/1
  g/1 -> Product/1
  Product/1 -> Sum1/2
  T_ld/1 -> Gain/1
  Gain4/1 -> Sin/1
  Gain3/1 -> Integrator/1
  Gain1/1 -> Sum1/3
  Sin/1 -> Gain2/1
  Gain/1 -> Sum1/1
  Gain2/1 -> Product/2
  Sum1/1 -> Sum/2
  T_m/1 -> Sum/1
  Sum/1 -> Gain3/1

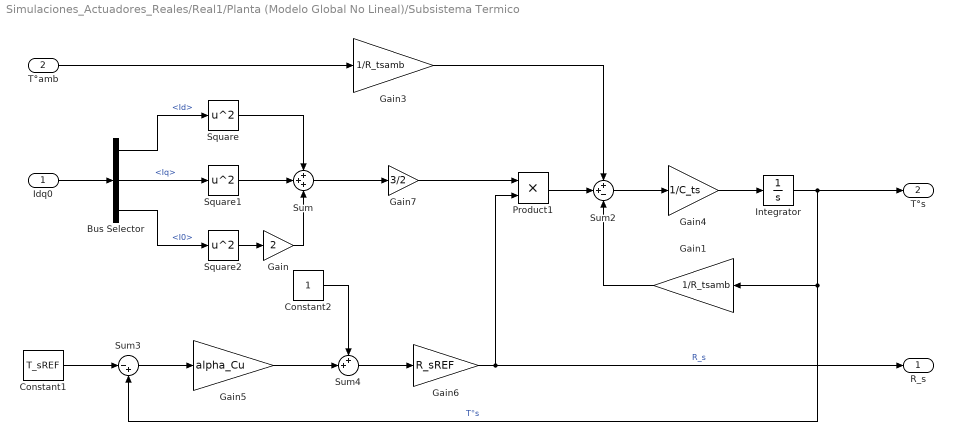
== system Simulaciones_Actuadores_Reales/Real1/Planta (Modelo Global No Lineal)/Subsistema Termico ==
  Idq0 : Inport
  T°amb : Inport  Port=2
  Bus Selector : BusSelector  OutputSignals=Id,Iq,I0
  Constant1 : Constant  Value=T_sREF
  Constant2 : Constant
  Gain : Gain  Gain=2
  Gain1 : Gain  Gain=1/R_tsamb
  Gain3 : Gain  Gain=1/R_tsamb
  Gain4 : Gain  Gain=1/C_ts
  Gain5 : Gain  Gain=alpha_Cu
  Gain6 : Gain  Gain=R_sREF
  Gain7 : Gain  Gain=3/2
  Integrator : Integrator  InitialCondition=init_Ts
  Product1 : Product
  Square : Math  Operator=square
  Square1 : Math  Operator=square
  Square2 : Math  Operator=square
  Sum : Sum  Inputs=+++
  Sum2 : Sum  Inputs=++-
  Sum3 : Sum  Inputs=|-+
  Sum4 : Sum  Inputs=++|
  R_s : Outport
  T°s : Outport  Port=2
  wires:
  Bus Selector/3 -> Square2/1  "<I0>"
  Bus Selector/1 -> Square/1  "<Id>"
  Constant2/1 -> Sum4/1
  Idq0/1 -> Bus Selector/1
  Gain3/1 -> Sum2/1
  Gain1/1 -> Sum2/3
  Gain4/1 -> Integrator/1
  Product1/1 -> Sum2/2
  Square/1 -> Sum/1
  Sum2/1 -> Gain4/1
  Square2/1 -> Gain/1
  Sum/1 -> Gain7/1
  T°amb/1 -> Gain3/1
  Sum3/1 -> Gain5/1
  Gain5/1 -> Sum4/2
  Gain/1 -> Sum/3
  Constant1/1 -> Sum3/1
  Sum4/1 -> Gain6/1
  Gain7/1 -> Product1/1
  Gain6/1 -> Product1/2, R_s/1  "R_s"
  Integrator/1 -> T°s/1, Gain1/1, Sum3/2  "T°s"
  Square1/1 -> Sum/2
  Bus Selector/2 -> Square1/1  "<Iq>"

== system Simulaciones_Actuadores_Reales/Real1/Subsystem Reference/Encoder- LP 2nd ==
  u : Inport
  Gain : Gain  Gain=wn_E^2
  Gain1 : Gain  Gain=wn_E^2
  Gain2 : Gain  Gain=2*zeta_E*wn_E
  Integrator : Integrator
  Integrator1 : Integrator
  Sum : Sum  Inputs=|++
  Sum1 : Sum  Inputs=|+-
  y : Outport
  wires:
  Integrator1/1 -> y/1, Gain1/1
  Integrator/1 -> Integrator1/1, Gain2/1
  Gain1/1 -> Sum/1
  Gain2/1 -> Sum/2
  Sum1/1 -> Integrator/1
  Sum/1 -> Sum1/2
  Gain/1 -> Sum1/1
  u/1 -> Gain/1

== system Simulaciones_Actuadores_Reales/Real1/Subsystem Reference/Sensor Ia - LP 2nd ==
  u : Inport
  Gain : Gain  Gain=wn_I^2
  Gain1 : Gain  Gain=wn_I^2
  Gain2 : Gain  Gain=2*zeta_I*wn_I
  Integrator : Integrator
  Integrator1 : Integrator
  Sum : Sum  Inputs=|++
  Sum1 : Sum  Inputs=|+-
  y : Outport
  wires:
  u/1 -> Gain/1
  Gain/1 -> Sum1/1
  Sum/1 -> Sum1/2
  Sum1/1 -> Integrator/1
  Gain2/1 -> Sum/2
  Gain1/1 -> Sum/1
  Integrator/1 -> Gain2/1, Integrator1/1
  Integrator1/1 -> Gain1/1, y/1

== system Simulaciones_Actuadores_Reales/Real1/Subsystem Reference/Sensor Ib - LP 2nd ==
  u : Inport
  Gain : Gain  Gain=wn_I^2
  Gain1 : Gain  Gain=wn_I^2
  Gain2 : Gain  Gain=2*zeta_I*wn_I
  Integrator : Integrator
  Integrator1 : Integrator
  Sum : Sum  Inputs=|++
  Sum1 : Sum  Inputs=|+-
  y : Outport
  wires:
  Integrator1/1 -> y/1, Gain1/1
  Integrator/1 -> Integrator1/1, Gain2/1
  Gain1/1 -> Sum/1
  Gain2/1 -> Sum/2
  Sum1/1 -> Integrator/1
  Sum/1 -> Sum1/2
  Gain/1 -> Sum1/1
  u/1 -> Gain/1

== system Simulaciones_Actuadores_Reales/Real1/Subsystem Reference/Sensor Ic - LP 2nd ==
  u : Inport
  Gain : Gain  Gain=wn_I^2
  Gain1 : Gain  Gain=wn_I^2
  Gain2 : Gain  Gain=2*zeta_I*wn_I
  Integrator : Integrator
  Integrator1 : Integrator
  Sum : Sum  Inputs=|++
  Sum1 : Sum  Inputs=|+-
  y : Outport
  wires:
  u/1 -> Gain/1
  Gain/1 -> Sum1/1
  Sum/1 -> Sum1/2
  Sum1/1 -> Integrator/1
  Gain2/1 -> Sum/2
  Gain1/1 -> Sum/1
  Integrator/1 -> Gain2/1, Integrator1/1
  Integrator1/1 -> Gain1/1, y/1

== system Simulaciones_Actuadores_Reales/Real1/Subsystem Reference/Sensor RTD - LP 1nd ==
  u : Inport
  Gain : Gain  Gain=1/tau_RTD
  Integrator : Integrator
  Sum1 : Sum  Inputs=|+-
  y : Outport
  wires:
  Sum1/1 -> Gain/1
  u/1 -> Sum1/1
  Integrator/1 -> Sum1/2, y/1
  Gain/1 -> Integrator/1

== system Simulaciones_Actuadores_Reales/Real1/Modulador de Torque Equivalente/Lazo de Control de Corrientes Virtuales/Transformada Directa de Park ==
  Iabc : Inport
  θm : Inport  Port=2
  Bus Creator : BusCreator  Inputs=3
  Demux : Demux  Outputs=3
  Gain3 : Gain  Gain=Pp
  Park Transform : eeTransforms/Park Transform  AxisAlignment=Q-axis  PowerInvariant=off
      settings: LibrarySourceBlock=|
      | ee_sl_lib/Mathematical
      | Transforms/Park Transform
  Idq0 : Outport
  wires:
  Gain3/1 -> Park Transform/2
  Park Transform/1 -> Demux/1  "Idq0"
  Demux/1 -> Bus Creator/1  "Id"
  Demux/3 -> Bus Creator/3  "I0"
  Demux/2 -> Bus Creator/2  "Iq"
  Bus Creator/1 -> Idq0/1
  Iabc/1 -> Park Transform/1
  θm/1 -> Gain3/1

== system Simulaciones_Actuadores_Reales/Real1/Modulador de Torque Equivalente/Modulador de Tensiones Virtuales/Subsystem Reference ==
  θm : Inport
  Vd : Inport  Port=2
  Vq : Inport  Port=3
  V0 : Inport  Port=4
  Bus Creator : BusCreator  Inputs=3
  Bus Creator1 : BusCreator  Inputs=3
  Demux : Demux  Outputs=3
  Gain3 : Gain  Gain=Pp
  Inverse Park Transform : eeTransforms/Inverse Park Transform  AxisAlignment=Q-axis  PowerInvariant=off
      settings: LibrarySourceBlock=|
      | ee_sl_lib/Mathematical
      | Transforms/Inverse
      | Park Transform
  Vdq0 : Outport
  Vabc : Outport  Port=2
  wires:
  Bus Creator1/1 -> Inverse Park Transform/1, Vdq0/1
  V0/1 -> Bus Creator1/3
  Vq/1 -> Bus Creator1/2
  Vd/1 -> Bus Creator1/1
  θm/1 -> Gain3/1
  Bus Creator/1 -> Vabc/1
  Demux/2 -> Bus Creator/2  "Vb"
  Demux/3 -> Bus Creator/3  "Vc"
  Demux/1 -> Bus Creator/1  "Va"
  Inverse Park Transform/1 -> Demux/1  "v_abc"
  Gain3/1 -> Inverse Park Transform/2

== system Simulaciones_Actuadores_Reales/Real1/Modulador de Torque Equivalente/Modulador de Tensiones Virtuales/Transformada Directa de Park ==
  Iabc : Inport
  θm : Inport  Port=2
  Bus Creator : BusCreator  Inputs=3
  Demux : Demux  Outputs=3
  Gain3 : Gain  Gain=Pp
  Park Transform : eeTransforms/Park Transform  AxisAlignment=Q-axis  PowerInvariant=off
      settings: LibrarySourceBlock=|
      | ee_sl_lib/Mathematical
      | Transforms/Park Transform
  Idq0 : Outport
  wires:
  θm/1 -> Gain3/1
  Iabc/1 -> Park Transform/1
  Bus Creator/1 -> Idq0/1
  Demux/2 -> Bus Creator/2  "Iq"
  Demux/3 -> Bus Creator/3  "I0"
  Demux/1 -> Bus Creator/1  "Id"
  Park Transform/1 -> Demux/1  "Idq0"
  Gain3/1 -> Park Transform/2

== system Simulaciones_Actuadores_Reales/Real1/Modulador de Torque Equivalente/Modulador y Compensación de Torque/Transformada Directa de Park ==
  θm : Inport
  Iabc : Inport  Port=2
  Bus Creator : BusCreator  Inputs=3
  Demux : Demux  Outputs=3
  Gain3 : Gain  Gain=Pp
  Park Transform : eeTransforms/Park Transform  AxisAlignment=Q-axis  PowerInvariant=off
      settings: LibrarySourceBlock=|
      | ee_sl_lib/Mathematical
      | Transforms/Park Transform
  Idq0 : Outport
  wires:
  Gain3/1 -> Park Transform/2
  Park Transform/1 -> Demux/1  "Idq0"
  Demux/1 -> Bus Creator/1  "Id"
  Demux/3 -> Bus Creator/3  "I0"
  Demux/2 -> Bus Creator/2  "Iq"
  Bus Creator/1 -> Idq0/1
  Iabc/1 -> Park Transform/1
  θm/1 -> Gain3/1
